simulink model "model"  (R2024b)
settings: Solver=VariableStepAuto  StartTime=0.0  StopTime=2000  RelTol=1e-3
values from neighbouring files (symbols this model uses):
  beta = 0.81    [setup_params.m]
  dist_profile_slope = [0, 3, 3 + tiny_step, 4, 4 + tiny_step, 8, 8 + tiny_step, 9, 9 + tiny_step, 10]    [setup_params.m]
  dist_profile_speed = [0, 1, 1 + tiny_step, 4, 4 + tiny_step, 6, 6 + tiny_step, 9, 9 + tiny_step, 10, 10 + tiny_step, final_stop_dist]    [setup_params.m]
  En = V_dc - (Ra * Iar)    (= 539.16)    [setup_params.m]
  Ier = 5    [setup_params.m]
  Jeq = 90.56    [setup_params.m]
  La = 0.0039    [setup_params.m]
  Le = 1.2    [setup_params.m]
  Omega_r_rads = Omega_r_rpm * (2*pi/60)    (= 101.578162466)    [setup_params.m]
  r = 0.34    [setup_params.m]
  Ra = 0.39    [setup_params.m]
  Re = 12    [setup_params.m]
  rho = 13/74    (= 0.175675675676)    [setup_params.m]
  slope_profile = [0, 0, 5, 5, 0, 0, -5, -5, 0, 0]    [setup_params.m]
  speed_req_kmh = [vr_kmh/2, vr_kmh/2, vr_kmh, vr_kmh, vmax_kmh, vmax_kmh, vr_kmh, vr_kmh, vr_kmh/2, vr_kmh/2, 0, 0]    [setup_params.m]
  V_dc = 600    [setup_params.m]
undefined symbols (not defined in the file or in its folder): C_speed
libraries: slpidlib x3
settings Model: Creator=Karim Negm  LastModifiedBy=Karim Negm

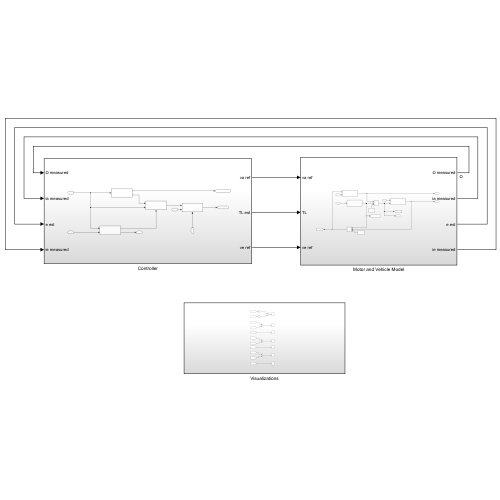
[thumbnail: Simulink's stored preview of the top-level diagram]
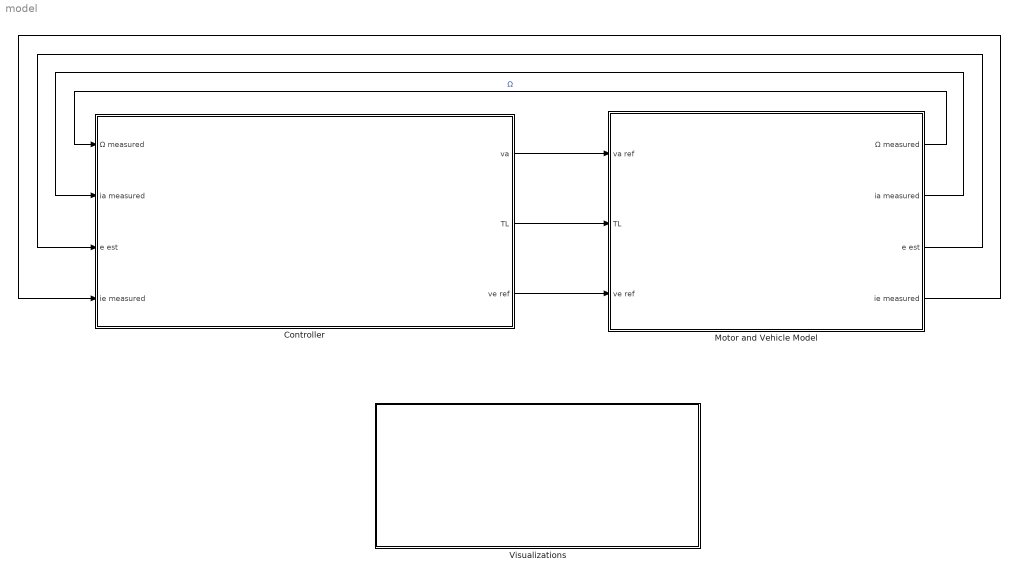
== system model ==
  Controller : Subsystem
  Motor and Vehicle Model : Subsystem
  Visualizations : Subsystem
  wires:
  Motor and Vehicle Model/2(ia measured) -> Controller/2(ia measured)
  Motor and Vehicle Model/3(e est) -> Controller/3(e est)
  Motor and Vehicle Model/4(ie measured) -> Controller/4(ie measured)
  Motor and Vehicle Model/1(Ω measured) -> Controller/1(Ω measured)  "Ω"
  Controller/1(va) -> Motor and Vehicle Model/1(va ref)
  Controller/2(TL) -> Motor and Vehicle Model/2(TL)
  Controller/3(ve ref) -> Motor and Vehicle Model/3(ve ref)

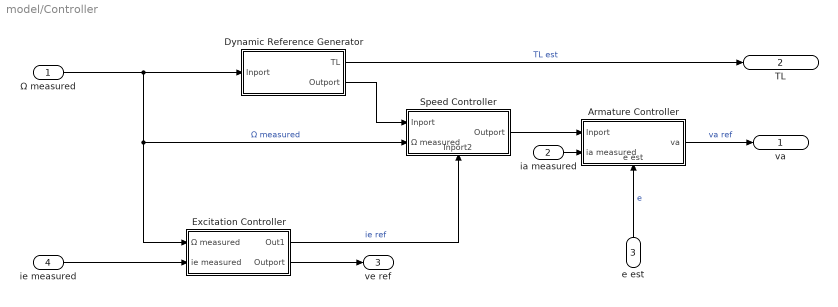
== system model/Controller ==
  Ω measured : Inport
  ia measured : Inport  Port=2
  e est : Inport  Port=3
  ie measured : Inport  Port=4
  Armature Controller : Subsystem
      settings: PortSchema="{\"entries\":[{\"content\":{\"sides\":[{\"content\":{\"connectorIds\":[\"In1\",\"In2\"]},\"type\":\"ConnectorPlacement.EquallySpacedRectSide\",\"uuid\":\"b1610dae-6d89-44cb-a946-9b88326d943b\"},{\"content\":{\"connectorIds\":[\"Out1\"],\"side\":\"RIGHT\"},\"type\":\"ConnectorPlacement.EquallySpacedRectSide\",\"uuid\":\"f41bd1e7-444e-410d-b339-c78692e6f3e8\"},{\"content\":{\"side\":\"TOP\"},\"type\":\"ConnectorPlacement.EquallySpacedRectSide\",\"uuid\":\"bb6f52aa-385e-4d07-b767-54f5b10ad36b\"},{\"content\":{\"connectorIds\":[\"In3\"],\"side\":\"BOTTOM\"},\"type\":\"ConnectorPlacement.EquallySpacedRectSide\",\"uuid\":\"26dba0af-1e42-4a62-99a9-c824ff2552de\"}]},\"type\":\"ConnectorPlacement.EquallySpacedConnector\",\"uuid\":\"cfe31124-8035-4304-a818-392152bdd9d8\"}],\"packageUris\":[\"http://schema.mathworks.com/mf0/Connector/R2020b\"],\"version\":\"1.0\"}"
  Dynamic Reference Generator : Subsystem
  Excitation Controller : Subsystem
  Speed Controller : Subsystem
      settings: PortSchema="{\"entries\":[{\"content\":{\"sides\":[{\"content\":{\"connectorIds\":[\"In1\",\"In2\"]},\"type\":\"ConnectorPlacement.EquallySpacedRectSide\",\"uuid\":\"b1610dae-6d89-44cb-a946-9b88326d943b\"},{\"content\":{\"connectorIds\":[\"Out1\"],\"side\":\"RIGHT\"},\"type\":\"ConnectorPlacement.EquallySpacedRectSide\",\"uuid\":\"f41bd1e7-444e-410d-b339-c78692e6f3e8\"},{\"content\":{\"side\":\"TOP\"},\"type\":\"ConnectorPlacement.EquallySpacedRectSide\",\"uuid\":\"bb6f52aa-385e-4d07-b767-54f5b10ad36b\"},{\"content\":{\"connectorIds\":[\"In3\"],\"side\":\"BOTTOM\"},\"type\":\"ConnectorPlacement.EquallySpacedRectSide\",\"uuid\":\"61bb23fc-2a87-4d69-b5d9-84aba53d439e\"}]},\"type\":\"ConnectorPlacement.EquallySpacedConnector\",\"uuid\":\"cfe31124-8035-4304-a818-392152bdd9d8\"}],\"packageUris\":[\"http://schema.mathworks.com/mf0/Connector/R2020b\"],\"version\":\"1.0\"}"
  va : Outport
  TL : Outport  Port=2
  ve ref : Outport  Port=3
  wires:
  Ω measured/1 -> Speed Controller/2(Ω measured), Excitation Controller/1(Ω measured), Dynamic Reference Generator/1(Inport)  "Ω measured"
  ie measured/1 -> Excitation Controller/2(ie measured)
  Excitation Controller/2(Outport) -> ve ref/1
  ia measured/1 -> Armature Controller/2(ia measured)
  e est/1 -> Armature Controller/3(e est)  "e"
  Armature Controller/1(va) -> va/1  "va ref"
  Speed Controller/1(Outport) -> Armature Controller/1(Inport)
  Excitation Controller/1(Out1) -> Speed Controller/3(Inport2)  "ie ref"
  Dynamic Reference Generator/2(Outport) -> Speed Controller/1(Inport)
  Dynamic Reference Generator/1(TL) -> TL/1  "TL est"

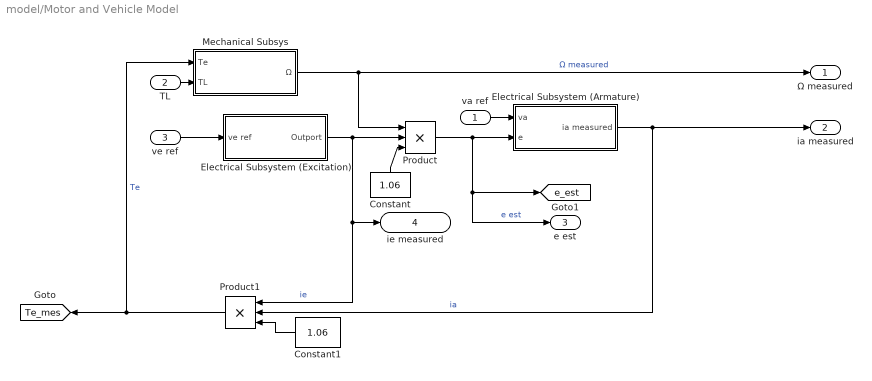
== system model/Motor and Vehicle Model ==
  va ref : Inport
  TL : Inport  Port=2
  ve ref : Inport  Port=3
  Constant : Constant  Value=1.06
  Constant1 : Constant  Value=1.06
  Electrical Subsystem (Armature) : Subsystem
  Electrical Subsystem (Excitation) : Subsystem
  Mechanical Subsys : Subsystem
  Product : Product  Inputs=3
  Product1 : Product  Inputs=3
  Ω measured : Outport
  ia measured : Outport  Port=2
  e est : Outport  Port=3
  ie measured : Outport  Port=4
  tag scope: Te_mes=global, e_est=global
  wires:
  Mechanical Subsys/1(Ω) -> Ω measured/1, Product/1  "Ω measured"
  Product/1 -> Electrical Subsystem (Armature)/2(e), e est/1, [e_est]  "e est"
  Electrical Subsystem (Armature)/1(ia measured) -> ia measured/1, Product1/2  "ia"
  Product1/1 -> Mechanical Subsys/1(Te), [Te_mes]  "Te"
  TL/1 -> Mechanical Subsys/2(TL)
  va ref/1 -> Electrical Subsystem (Armature)/1(va)
  Electrical Subsystem (Excitation)/1(Outport) -> Product/2, Product1/1, ie measured/1  "ie"
  ve ref/1 -> Electrical Subsystem (Excitation)/1(ve ref)
  Constant/1 -> Product/3
  Constant1/1 -> Product1/3

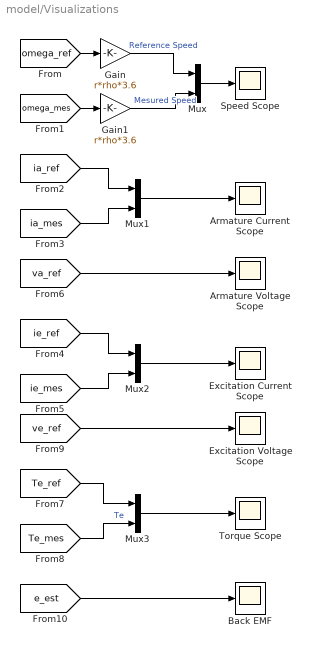
== system model/Visualizations ==
  Armature Current Scope : Scope
  Armature Voltage Scope : Scope
  Back EMF : Scope
  Excitation Current Scope : Scope
  Excitation Voltage Scope : Scope
  Gain : Gain  Gain=r*rho*3.6
  Gain1 : Gain  Gain=r*rho*3.6
  Mux{,1..3} (4 alike) : Mux  Inputs=2
  Speed Scope : Scope
  Torque Scope : Scope
  wires:
  Mux/1 -> Speed Scope/1
  Mux1/1 -> Armature Current Scope/1
  [ia_mes] -> Mux1/2
  [ia_ref] -> Mux1/1
  Mux2/1 -> Excitation Current Scope/1
  [ie_ref] -> Mux2/1
  [ie_mes] -> Mux2/2
  [va_ref] -> Armature Voltage Scope/1
  Mux3/1 -> Torque Scope/1
  [Te_ref] -> Mux3/1
  [Te_mes] -> Mux3/2  "Te"
  [ve_ref] -> Excitation Voltage Scope/1
  [e_est] -> Back EMF/1
  [omega_mes] -> Gain1/1
  [omega_ref] -> Gain/1
  Gain/1 -> Mux/1  "Reference Speed"
  Gain1/1 -> Mux/2  "Mesured Speed"

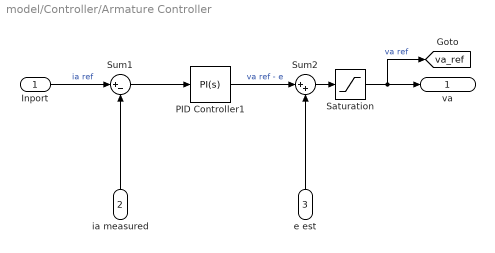
== system model/Controller/Armature Controller ==
  Inport : Inport
  ia measured : Inport  Port=2
  e est : Inport  Port=3
  PID Controller1 : slpidlib/PID Controller  Controller=PI  Form=Parallel  TimeDomain=Continuous-time  UseExternalTs=off  SampleTime=-1  IntegratorMethod=Forward Euler  FilterMethod=Forward Euler  ControllerParametersSource=internal  P=7.8  I=78  UseKiTs=off  D=0  UseExternalDerivativeSource=off  N=100  UseFilter=on  TunerSelectOption=Transfer Function Based (PID Tuner App)  ZeroCross=off  InitialConditionSource=internal  InitialConditionForIntegrator=0  InitialConditionForFilter=0  DifferentiatorICPrevScaledInput=0  ExternalReset=none  TrackingMode=off  Kt=1  LimitOutput=on  SatLimitsSource=internal  UpperSaturationLimit=V_dc - En  LowerSaturationLimit=-(V_dc - En)  LinearizeAsGain=on  AntiWindupMode=back-calculation  Kb=1  LimitIntegrator=off  UpperIntegratorSaturationLimit=inf  LowerIntegratorSaturationLimit=-inf  POutMin=[]  POutMax=[]  IOutMin=[]  IOutMax=[]  DOutMin=[]  DOutMax=[]  NOutMin=[]  NOutMax=[]  SumOutMin=[]  SumOutMax=[]  SaturationOutMin=[]  SaturationOutMax=[]  PParamMin=[]  PParamMax=[]  IParamMin=[]  IParamMax=[]  DParamMin=[]  DParamMax=[]  NParamMin=[]  NParamMax=[]  KbParamMin=[]  KbParamMax=[]  KtParamMin=[]  KtParamMax=[]  KbOutMin=[]  KbOutMax=[]  KtOutMin=[]  KtOutMax=[]  IntegratorOutMin=[]  IntegratorOutMax=[]  FilterOutMin=[]  FilterOutMax=[]  SumI1OutMin=[]  SumI1OutMax=[]  SumI2OutMin=[]  SumI2OutMax=[]  SumI3OutMin=[]  SumI3OutMax=[]  SumI4OutMin=[]  SumI4OutMax=[]  SumDOutMin=[]  SumDOutMax=[]  DifferentiatorOutMin=[]  DifferentiatorOutMax=[]  FilterDiffOutCoefMin=[]  FilterDiffOutCoefMax=[]  ReciprocalOutMin=[]  ReciprocalOutMax=[]  SumDenOutMin=[]  SumDenOutMax=[]  SumNumOutMin=[]  SumNumOutMax=[]  DivideOutMin=[]  DivideOutMax=[]  UdiffTsProdOutMin=[]  UdiffTsProdOutMax=[]  NTsProdOutMin=[]  NTsProdOutMax=[]  UintegralTsProdOutMin=[]  UintegralTsProdOutMax=[]  UngainTsProdOutMin=[]  UngainTsProdOutMax=[]  ClampingZeroOutDataTypeStr=Inherit: Inherit via back propagation  ClampingZeroOutMin=[]  ClampingZeroOutMax=[]  FilterDenConstantOutDataTypeStr=Inherit: Inherit via back propagation  FilterDenConstantOutMin=[]  FilterDenConstantOutMax=[]  PCopyOutDataTypeStr=Inherit: Inherit via back propagation  PCopyOutMin=[]  PCopyOutMax=[]  NCopyOutDataTypeStr=Inherit: Inherit via back propagation  NCopyOutMin=[]  NCopyOutMax=[]  IntegratorContinuousStateAttributes=''  IntegratorStateMustResolveToSignalObject=off  IntegratorRTWStateStorageClass=Auto  FilterContinuousStateAttributes=''  FilterStateMustResolveToSignalObject=off  FilterRTWStateStorageClass=Auto  ParallelPVariant=InternalParameters  IdealPVariant=Disabled  IVariant=InternalParameters  DVariant=Disabled  IntegratorVariant=Continuous  SatVariant=Enabled  AWVariant=BackCalculation  PCopyVariant=Disabled  TRVariant=Disabled  FdbkBlocksVariant=Forward  IdealPFdbkVariant=Disabled  SatFdbkVariant=Disabled  DerivativeFilterVariant=Disabled  NVariant=Disabled  NCopyVariant=Disabled_SignalSpec  FilterICVariant=Disabled  IntegratorICVariant=InternalICs  ExternalResetVariant=Disabled  TRSumVariant=Passthrough  SumFdbkVariant=Disabled  SumVariant=Sum_PI  TsampFilterVariant=InternalTs  TsampNgainVariant=Passthrough  TsampIntegralVariant=Disabled_SignalSpec  ExternalSaturationOutDataTypeStr=Inherit: Same as second input  DerivativeSourceVariant=Disabled  PreIntVariant=InternalPreInt
  Saturation : Saturate  UpperLimit=600  LowerLimit=-600
  Sum1 : Sum  Inputs=|+-
  Sum2 : Sum  Inputs=|++
  va : Outport
  tag scope: va_ref=global
  wires:
  Inport/1 -> Sum1/1  "ia ref"
  ia measured/1 -> Sum1/2
  Sum1/1 -> PID Controller1/1
  e est/1 -> Sum2/2
  PID Controller1/1 -> Sum2/1  "va ref - e"
  Sum2/1 -> Saturation/1
  Saturation/1 -> [va_ref], va/1  "va ref"

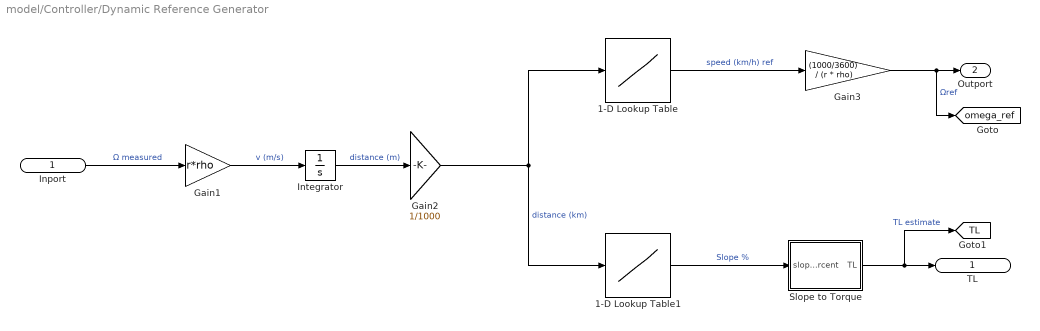
== system model/Controller/Dynamic Reference Generator ==
  Inport : Inport
  1-D Lookup Table : Lookup_n-D  NumberOfTableDimensions=1  BreakpointsForDimension1=dist_profile_speed  Table=speed_req_kmh  InternalRulePriority=Speed  RndMeth=Simplest
  1-D Lookup Table1 : Lookup_n-D  NumberOfTableDimensions=1  BreakpointsForDimension1=dist_profile_slope  Table=slope_profile  InternalRulePriority=Speed  RndMeth=Simplest
  Gain1 : Gain  Gain=r*rho
  Gain2 : Gain  Gain=1/1000
  Gain3 : Gain  Gain=(1000/3600) / (r * rho)
  Integrator : Integrator
  "Slope to Torque " : MATLAB Function  TreatAsAtomicUnit=on
  TL : Outport
  Outport : Outport  Port=2
  tag scope: TL=global, omega_ref=global
  wires:
  1-D Lookup Table/1 -> Gain3/1  "speed (km/h) ref"
  "Slope to Torque "/1(TL) -> [TL], TL/1  "TL estimate"
  1-D Lookup Table1/1 -> "Slope to Torque "/1(slope_percent)  "Slope %"
  Integrator/1 -> Gain2/1  "distance (m)"
  Gain2/1 -> 1-D Lookup Table1/1, 1-D Lookup Table/1  "distance (km)"
  Gain1/1 -> Integrator/1  "v (m/s)"
  Inport/1 -> Gain1/1  "Ω measured"
  Gain3/1 -> [omega_ref], Outport/1  "Ωref"

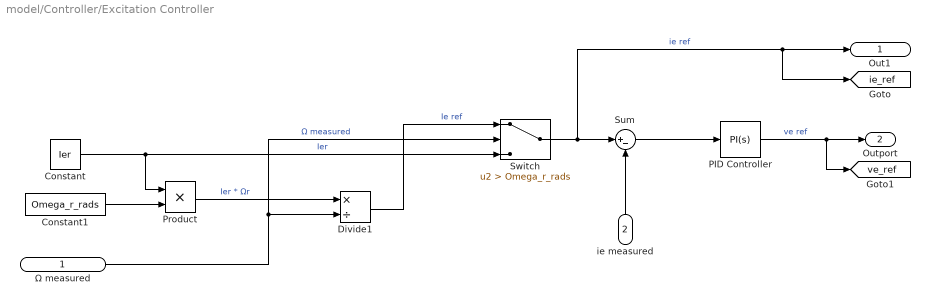
== system model/Controller/Excitation Controller ==
  Ω measured : Inport
  ie measured : Inport  Port=2
  Constant : Constant  Value=Ier
  Constant1 : Constant  Value=Omega_r_rads
  Divide1 : Product  Inputs=*/
  PID Controller : slpidlib/PID Controller  Controller=PI  Form=Parallel  TimeDomain=Continuous-time  UseExternalTs=off  SampleTime=-1  IntegratorMethod=Forward Euler  FilterMethod=Forward Euler  ControllerParametersSource=internal  P=24  I=240  UseKiTs=off  D=0  UseExternalDerivativeSource=off  N=100  UseFilter=on  TunerSelectOption=Transfer Function Based (PID Tuner App)  ZeroCross=off  InitialConditionSource=internal  InitialConditionForIntegrator=0  InitialConditionForFilter=0  DifferentiatorICPrevScaledInput=0  ExternalReset=none  TrackingMode=off  Kt=1  LimitOutput=on  SatLimitsSource=internal  UpperSaturationLimit=60  LowerSaturationLimit=-60  LinearizeAsGain=on  AntiWindupMode=back-calculation  Kb=1  LimitIntegrator=off  UpperIntegratorSaturationLimit=inf  LowerIntegratorSaturationLimit=-inf  POutMin=[]  POutMax=[]  IOutMin=[]  IOutMax=[]  DOutMin=[]  DOutMax=[]  NOutMin=[]  NOutMax=[]  SumOutMin=[]  SumOutMax=[]  SaturationOutMin=[]  SaturationOutMax=[]  PParamMin=[]  PParamMax=[]  IParamMin=[]  IParamMax=[]  DParamMin=[]  DParamMax=[]  NParamMin=[]  NParamMax=[]  KbParamMin=[]  KbParamMax=[]  KtParamMin=[]  KtParamMax=[]  KbOutMin=[]  KbOutMax=[]  KtOutMin=[]  KtOutMax=[]  IntegratorOutMin=[]  IntegratorOutMax=[]  FilterOutMin=[]  FilterOutMax=[]  SumI1OutMin=[]  SumI1OutMax=[]  SumI2OutMin=[]  SumI2OutMax=[]  SumI3OutMin=[]  SumI3OutMax=[]  SumI4OutMin=[]  SumI4OutMax=[]  SumDOutMin=[]  SumDOutMax=[]  DifferentiatorOutMin=[]  DifferentiatorOutMax=[]  FilterDiffOutCoefMin=[]  FilterDiffOutCoefMax=[]  ReciprocalOutMin=[]  ReciprocalOutMax=[]  SumDenOutMin=[]  SumDenOutMax=[]  SumNumOutMin=[]  SumNumOutMax=[]  DivideOutMin=[]  DivideOutMax=[]  UdiffTsProdOutMin=[]  UdiffTsProdOutMax=[]  NTsProdOutMin=[]  NTsProdOutMax=[]  UintegralTsProdOutMin=[]  UintegralTsProdOutMax=[]  UngainTsProdOutMin=[]  UngainTsProdOutMax=[]  ClampingZeroOutDataTypeStr=Inherit: Inherit via back propagation  ClampingZeroOutMin=[]  ClampingZeroOutMax=[]  FilterDenConstantOutDataTypeStr=Inherit: Inherit via back propagation  FilterDenConstantOutMin=[]  FilterDenConstantOutMax=[]  PCopyOutDataTypeStr=Inherit: Inherit via back propagation  PCopyOutMin=[]  PCopyOutMax=[]  NCopyOutDataTypeStr=Inherit: Inherit via back propagation  NCopyOutMin=[]  NCopyOutMax=[]  IntegratorContinuousStateAttributes=''  IntegratorStateMustResolveToSignalObject=off  IntegratorRTWStateStorageClass=Auto  FilterContinuousStateAttributes=''  FilterStateMustResolveToSignalObject=off  FilterRTWStateStorageClass=Auto  ParallelPVariant=InternalParameters  IdealPVariant=Disabled  IVariant=InternalParameters  DVariant=Disabled  IntegratorVariant=Continuous  SatVariant=Enabled  AWVariant=BackCalculation  PCopyVariant=Disabled  TRVariant=Disabled  FdbkBlocksVariant=Forward  IdealPFdbkVariant=Disabled  SatFdbkVariant=Disabled  DerivativeFilterVariant=Disabled  NVariant=Disabled  NCopyVariant=Disabled_SignalSpec  FilterICVariant=Disabled  IntegratorICVariant=InternalICs  ExternalResetVariant=Disabled  TRSumVariant=Passthrough  SumFdbkVariant=Disabled  SumVariant=Sum_PI  TsampFilterVariant=InternalTs  TsampNgainVariant=Passthrough  TsampIntegralVariant=Disabled_SignalSpec  ExternalSaturationOutDataTypeStr=Inherit: Same as second input  DerivativeSourceVariant=Disabled  PreIntVariant=InternalPreInt
  Product : Product
  Sum : Sum  Inputs=|+-
  Switch : Switch  Criteria=u2 > Threshold  Threshold=Omega_r_rads  SaturateOnIntegerOverflow=off  InputSameDT=off
  Out1 : Outport
  Outport : Outport  Port=2
  tag scope: ie_ref=global, ve_ref=global
  wires:
  Ω measured/1 -> Switch/2, Divide1/2  "Ω measured"
  Constant/1 -> Product/1, Switch/3  "Ier"
  Product/1 -> Divide1/1  "Ier * Ωr"
  Constant1/1 -> Product/2
  Divide1/1 -> Switch/1  "Ie ref"
  Sum/1 -> PID Controller/1
  PID Controller/1 -> [ve_ref], Outport/1  "ve ref"
  ie measured/1 -> Sum/2
  Switch/1 -> [ie_ref], Out1/1, Sum/1  "ie ref"

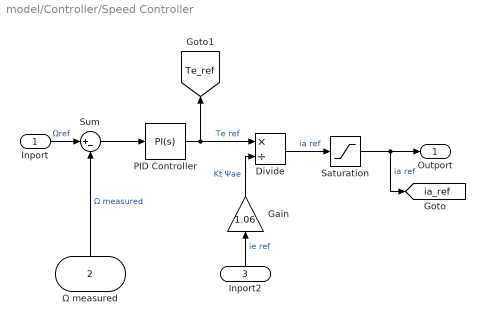
== system model/Controller/Speed Controller ==
  Inport : Inport
  Ω measured : Inport  Port=2
  Inport2 : Inport  Port=3
  Divide : Product  Inputs=*/
  Gain : Gain  Gain=1.06
  PID Controller : slpidlib/PID Controller  Controller=PI  Form=Parallel  TimeDomain=Continuous-time  UseExternalTs=off  SampleTime=-1  IntegratorMethod=Forward Euler  FilterMethod=Forward Euler  ControllerParametersSource=internal  P=C_speed.Kp  I=C_speed.Ki  UseKiTs=off  D=0  UseExternalDerivativeSource=off  N=100  UseFilter=on  TunerSelectOption=Transfer Function Based (PID Tuner App)  InitialConditionSource=internal  InitialConditionForIntegrator=0  InitialConditionForFilter=0  DifferentiatorICPrevScaledInput=0  ExternalReset=none  TrackingMode=off  Kt=1  LimitOutput=on  SatLimitsSource=internal  UpperSaturationLimit=830  LowerSaturationLimit=-830  LinearizeAsGain=on  AntiWindupMode=back-calculation  Kb=1  LimitIntegrator=off  UpperIntegratorSaturationLimit=inf  LowerIntegratorSaturationLimit=-inf  POutMin=[]  POutMax=[]  IOutMin=[]  IOutMax=[]  DOutMin=[]  DOutMax=[]  NOutMin=[]  NOutMax=[]  SumOutMin=[]  SumOutMax=[]  SaturationOutMin=[]  SaturationOutMax=[]  PParamMin=[]  PParamMax=[]  IParamMin=[]  IParamMax=[]  DParamMin=[]  DParamMax=[]  NParamMin=[]  NParamMax=[]  KbParamMin=[]  KbParamMax=[]  KtParamMin=[]  KtParamMax=[]  KbOutMin=[]  KbOutMax=[]  KtOutMin=[]  KtOutMax=[]  IntegratorOutMin=[]  IntegratorOutMax=[]  FilterOutMin=[]  FilterOutMax=[]  SumI1OutMin=[]  SumI1OutMax=[]  SumI2OutMin=[]  SumI2OutMax=[]  SumI3OutMin=[]  SumI3OutMax=[]  SumI4OutMin=[]  SumI4OutMax=[]  SumDOutMin=[]  SumDOutMax=[]  DifferentiatorOutMin=[]  DifferentiatorOutMax=[]  FilterDiffOutCoefMin=[]  FilterDiffOutCoefMax=[]  ReciprocalOutMin=[]  ReciprocalOutMax=[]  SumDenOutMin=[]  SumDenOutMax=[]  SumNumOutMin=[]  SumNumOutMax=[]  DivideOutMin=[]  DivideOutMax=[]  UdiffTsProdOutMin=[]  UdiffTsProdOutMax=[]  NTsProdOutMin=[]  NTsProdOutMax=[]  UintegralTsProdOutMin=[]  UintegralTsProdOutMax=[]  UngainTsProdOutMin=[]  UngainTsProdOutMax=[]  ClampingZeroOutDataTypeStr=Inherit: Inherit via back propagation  ClampingZeroOutMin=[]  ClampingZeroOutMax=[]  FilterDenConstantOutDataTypeStr=Inherit: Inherit via back propagation  FilterDenConstantOutMin=[]  FilterDenConstantOutMax=[]  PCopyOutDataTypeStr=Inherit: Inherit via back propagation  PCopyOutMin=[]  PCopyOutMax=[]  NCopyOutDataTypeStr=Inherit: Inherit via back propagation  NCopyOutMin=[]  NCopyOutMax=[]  IntegratorContinuousStateAttributes=''  IntegratorStateMustResolveToSignalObject=off  IntegratorRTWStateStorageClass=Auto  FilterContinuousStateAttributes=''  FilterStateMustResolveToSignalObject=off  FilterRTWStateStorageClass=Auto  ParallelPVariant=InternalParameters  IdealPVariant=Disabled  IVariant=InternalParameters  DVariant=Disabled  IntegratorVariant=Continuous  SatVariant=Enabled  AWVariant=BackCalculation  PCopyVariant=Disabled  TRVariant=Disabled  FdbkBlocksVariant=Forward  IdealPFdbkVariant=Disabled  SatFdbkVariant=Disabled  DerivativeFilterVariant=Disabled  NVariant=Disabled  NCopyVariant=Disabled_SignalSpec  FilterICVariant=Disabled  IntegratorICVariant=InternalICs  ExternalResetVariant=Disabled  TRSumVariant=Passthrough  SumFdbkVariant=Disabled  SumVariant=Sum_PI  TsampFilterVariant=InternalTs  TsampNgainVariant=Passthrough  TsampIntegralVariant=Disabled_SignalSpec  ExternalSaturationOutDataTypeStr=Inherit: Same as second input  DerivativeSourceVariant=Disabled  PreIntVariant=InternalPreInt
  Saturation : Saturate  UpperLimit=156  LowerLimit=-156
  Sum : Sum  Inputs=|+-
  Outport : Outport
  tag scope: Te_ref=global, ia_ref=global
  wires:
  Inport2/1 -> Gain/1  "ie ref"
  PID Controller/1 -> Divide/1, [Te_ref]  "Te ref"
  Gain/1 -> Divide/2  "Kt Ψae"
  Inport/1 -> Sum/1  "Ωref"
  Ω measured/1 -> Sum/2  "Ω measured"
  Sum/1 -> PID Controller/1
  Divide/1 -> Saturation/1  "ia ref"
  Saturation/1 -> [ia_ref], Outport/1  "ia ref"

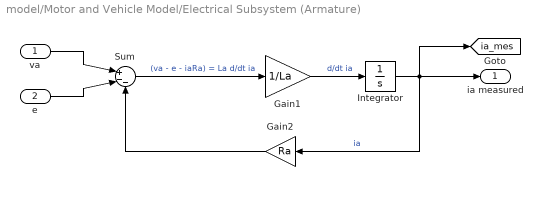
== system model/Motor and Vehicle Model/Electrical Subsystem (Armature) ==
  va : Inport
  e : Inport  Port=2
  Gain1 : Gain  Gain=1/La
  Gain2 : Gain  Gain=Ra
  Integrator : Integrator
  Sum : Sum  Inputs=|+--
  ia measured : Outport
  tag scope: ia_mes=global
  wires:
  va/1 -> Sum/1
  e/1 -> Sum/2
  Sum/1 -> Gain1/1  "(va - e - iaRa) = La d/dt ia"
  Gain1/1 -> Integrator/1  "d/dt ia"
  Integrator/1 -> [ia_mes], ia measured/1, Gain2/1  "ia"
  Gain2/1 -> Sum/3

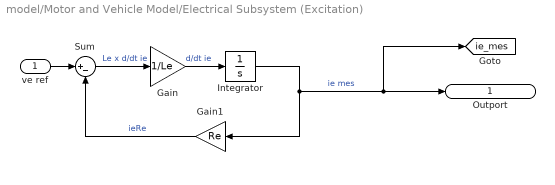
== system model/Motor and Vehicle Model/Electrical Subsystem (Excitation) ==
  ve ref : Inport
  Gain : Gain  Gain=1/Le
  Gain1 : Gain  Gain=Re
  Integrator : Integrator
  Sum : Sum  Inputs=|+-
  Outport : Outport
  tag scope: ie_mes=global
  wires:
  Gain1/1 -> Sum/2  "ieRe"
  Gain/1 -> Integrator/1  "d/dt ie"
  ve ref/1 -> Sum/1
  Sum/1 -> Gain/1  "Le x d/dt ie"
  Integrator/1 -> [ie_mes], Outport/1, Gain1/1  "ie mes"

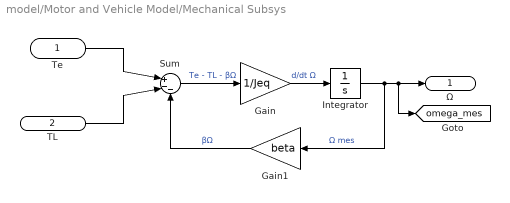
== system model/Motor and Vehicle Model/Mechanical Subsys ==
  Te : Inport
  TL : Inport  Port=2
  Gain : Gain  Gain=1/Jeq
  Gain1 : Gain  Gain=beta
  Integrator : Integrator
  Sum : Sum  Inputs=|+--
  Ω : Outport
  tag scope: omega_mes=global
  wires:
  Te/1 -> Sum/1
  Sum/1 -> Gain/1  "Te - TL - βΩ"
  Gain/1 -> Integrator/1  "d/dt Ω"
  Integrator/1 -> [omega_mes], Ω/1, Gain1/1  "Ω mes"
  TL/1 -> Sum/2
  Gain1/1 -> Sum/3  "βΩ"

== matlab function model/Controller/Dynamic Reference Generator/Slope to Torque  ==
  data: slope_percent input; TL output
function TL = fcn(slope_percent)
    M = 25400;
    g = 9.81;
    r = 0.34;
    rho = 13/74;

    theta = atan(slope_percent / 100);
    F_slope = M * g * sin(theta);
    T_wheel = F_slope * r;
    TL = T_wheel * rho;
end
